simulink model "Inversor_Ideal"  (R2026b)
settings: Solver=VariableStepAuto
settings Model: Creator=fedeb  LastModifiedBy=fedeb

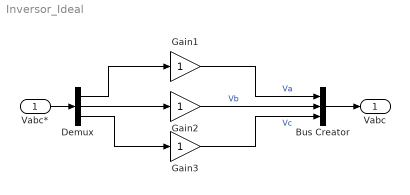
== system Inversor_Ideal ==
  Vabc* : Inport
  Bus Creator : BusCreator  Inputs=3
  Demux : Demux  Outputs=3
  Gain1 : Gain
  Gain2 : Gain
  Gain3 : Gain
  Vabc : Outport
  wires:
  Gain1/1 -> Bus Creator/1  "Va"
  Gain3/1 -> Bus Creator/3  "Vc"
  Bus Creator/1 -> Vabc/1
  Vabc*/1 -> Demux/1
  Demux/1 -> Gain1/1
  Gain2/1 -> Bus Creator/2  "Vb"
  Demux/3 -> Gain3/1
  Demux/2 -> Gain2/1
